simulink model "s20260910_config2torque_sim_pressure_torque"  (R2025a)
settings: Solver=VariableStepAuto  StartTime=0.0  StopTime=20  FixedStep=0.01  RelTol=1e-3  AbsTol=1e-3  EnableMultiTasking=on
undefined symbols (not defined in the file or in its folder): X, Y, Z
libraries: sm_lib x9, nesl_utility x4, cstblocks x2, snake_single_module_library_torque x1, slpidlib x1, simulink x1, snake_single_module_library_torque_multi x1
settings Model: Creator=dperera  LastModifiedBy=dperera
settings SolverCC: AutoScaleAbsTol=off  AlgebraicLoopSolver=TrustRegion  MaxZcPerStep=1.0
settings DataIOCC: LimitDataPoints=on  MaxDataPoints=10000
settings OptimizationCC: ReuseModelBlockBuffer=off  LifeSpan=inf
settings DebuggingCC: UnconnectedInputMsg=warning  UnconnectedOutputMsg=warning  UnconnectedLineMsg=warning  AllowSymbolicDim=off  SubsystemReferenceDiagnosticForUnitTest=warning  SFUnexpectedBacktrackingDiag=warning  SFNoUnconditionalDefaultTransitionDiag=warning  SFExecutionAtInitializationDiag=none  ArithmeticOperatorsInVariantConditions=warning
settings ModelReferenceCC: EnableRefExpFcnMdlSchedulingChecks=on
settings SFSimCC: SimUseLocalCustomCode=off  CustomCodeUndefinedFunction=UseInterfaceOnly
settings RTWCC: RTWUseLocalCustomCode=off  GPUComputeCapability=3.5  DLArmComputeVersion=19.05
settings CodeAppCC: StateflowObjectComments=on
settings GRTTargetCC: TargetLangStandard=C89/C90 (ANSI)
settings ConfigComp: CovMetricSettings=dw  CovSaveCumulativeToWorkspaceVar=on  CovSaveSingleToWorkspaceVar=on  CovExternalEMLEnable=off  CovSFcnEnable=off
settings SimscapeCC: SimscapeLogType=all  SimscapeLogSimulationStatistics=on  SimscapeLogDataHistory=10000.0

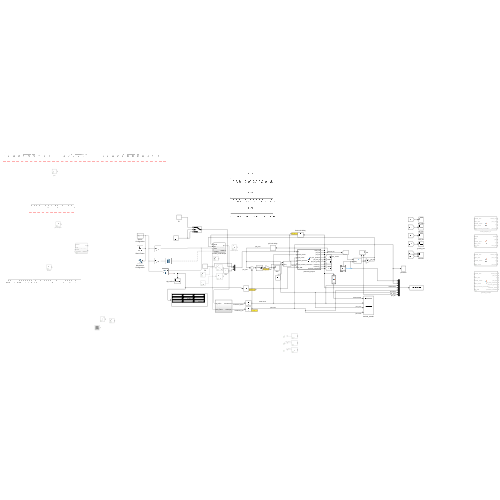
[thumbnail: Simulink's stored preview of the top-level diagram]
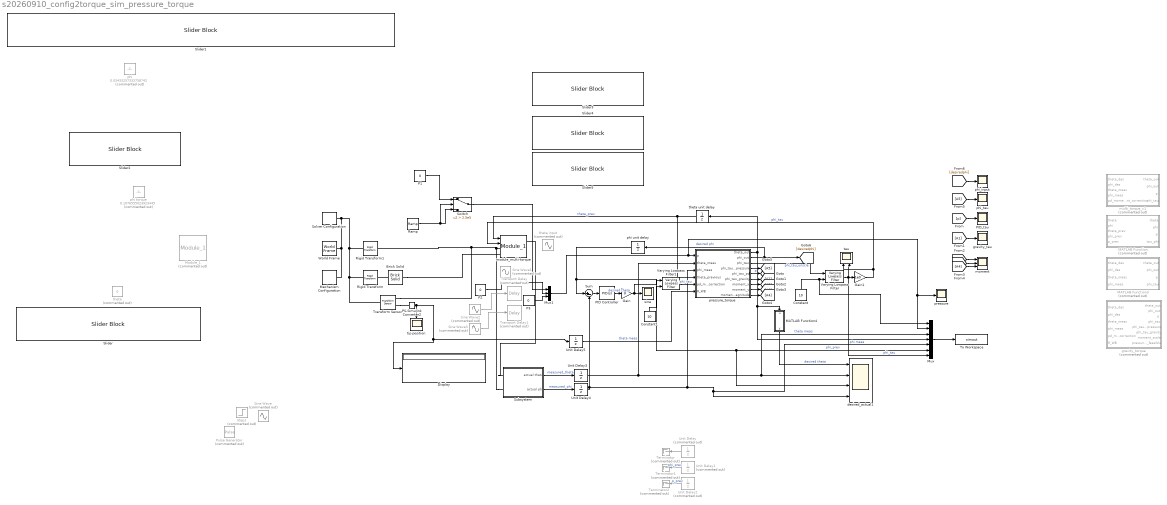
== system s20260910_config2torque_sim_pressure_torque ==
  Brick Solid : sm_lib/Body Elements/Brick Solid  BrickDimensions=[0.5 0.5 0.01]  BrickDimensionsUnits=m  ExportEntireGeometry=on  InertiaType=CalculateFromGeometry  BasedOnType=Density  Density=1000  DensityUnits=kg/m^3  Mass=1  MassUnits=kg  CenterOfMass=[0 0 0]  CenterOfMassUnits=m  MomentsOfInertia=[1 1 1]  MomentsOfInertiaUnits=kg*m^2  ProductsOfInertia=[0 0 0]  ProductsOfInertiaUnits=kg*m^2  GraphicType=FromGeometry  MarkerShape=Sphere  MarkerSize=10  GraphicVisPropType=SimpleVisualProperties  GraphicDiffuseColor=[0.5 0.5 0.5]  GraphicOpacity=1  GraphicSpecularColor=[0.5 0.5 0.5 1.0]  GraphicAmbientColor=[0.15 0.15 0.15 1.0]  GraphicEmissiveColor=[0.0 0.0 0.0 1.0]  GraphicShininess=75  DoExposeReferenceFrame=on  SerializedFrames=<Frames/>
  Constant : Constant  Value=10
  Constant1 : Constant  Value=10
  Display : Display
  Gain : Gain  Gain=0
  Gain1 : Gain  Gain=1e0
  MATLAB Function : MATLAB Function  Commented=on  TreatAsAtomicUnit=on
  MATLAB Function3 : MATLAB Function  Commented=on  TreatAsAtomicUnit=on
  MATLAB Function4 : MATLAB Function  TreatAsAtomicUnit=on
  Mechanism Configuration : sm_lib/Utilities/Mechanism Configuration  UniformGravity=Constant  GravityVector=[0 0 -9.80665]  GravityVectorUnits=m/s^2  LinearizationDelta=0.001  JointModeTransitionNonlinearIterations=2
  Module_1 : snake_single_module_library_torque/Module_1  Commented=on  SystemSampleTime=-1  VariantActivationTime=update diagram  EmptyChoice=off  PassThrough=off  PassThroughVariantControl=(default)  EmptyChoiceVariantControl=(default)  AllowFlexibleInterface=on  Latency=0  AutoFrameSizeCalculation=off
  Mux : Mux  Inputs=7
  Mux1 : Mux  Inputs=3
  P1 : Constant  Value=0
  P2 : Constant  Value=0
  P3 : Constant  Value=0
  PID Controller : slpidlib/PID Controller  Controller=PID  Form=Parallel  TimeDomain=Continuous-time  UseExternalTs=off  SampleTime=-1  IntegratorMethod=Forward Euler  FilterMethod=Forward Euler  ControllerParametersSource=internal  P=0.1  I=0.1  UseKiTs=off  D=0.0005  UseExternalDerivativeSource=off  N=100  UseFilter=on  TunerSelectOption=Frequency Response Based  InitialConditionSource=internal  InitialConditionForIntegrator=0  InitialConditionForFilter=0  DifferentiatorICPrevScaledInput=0  ExternalReset=none  TrackingMode=off  Kt=1  LimitOutput=on  SatLimitsSource=internal  UpperSaturationLimit=inf  LowerSaturationLimit=-inf  LinearizeAsGain=on  AntiWindupMode=back-calculation  Kb=1  LimitIntegrator=off  UpperIntegratorSaturationLimit=inf  LowerIntegratorSaturationLimit=-inf  POutMin=[]  POutMax=[]  IOutMin=[]  IOutMax=[]  DOutMin=[]  DOutMax=[]  NOutMin=[]  NOutMax=[]  SumOutMin=[]  SumOutMax=[]  SaturationOutMin=[]  SaturationOutMax=[]  PParamMin=[]  PParamMax=[]  IParamMin=[]  IParamMax=[]  DParamMin=[]  DParamMax=[]  NParamMin=[]  NParamMax=[]  KbParamMin=[]  KbParamMax=[]  KtParamMin=[]  KtParamMax=[]  KbOutMin=[]  KbOutMax=[]  KtOutMin=[]  KtOutMax=[]  IntegratorOutMin=[]  IntegratorOutMax=[]  FilterOutMin=[]  FilterOutMax=[]  SumI1OutMin=[]  SumI1OutMax=[]  SumI2OutMin=[]  SumI2OutMax=[]  SumI3OutMin=[]  SumI3OutMax=[]  SumI4OutMin=[]  SumI4OutMax=[]  SumDOutMin=[]  SumDOutMax=[]  DifferentiatorOutMin=[]  DifferentiatorOutMax=[]  FilterDiffOutCoefMin=[]  FilterDiffOutCoefMax=[]  ReciprocalOutMin=[]  ReciprocalOutMax=[]  SumDenOutMin=[]  SumDenOutMax=[]  SumNumOutMin=[]  SumNumOutMax=[]  DivideOutMin=[]  DivideOutMax=[]  UdiffTsProdOutMin=[]  UdiffTsProdOutMax=[]  NTsProdOutMin=[]  NTsProdOutMax=[]  UintegralTsProdOutMin=[]  UintegralTsProdOutMax=[]  UngainTsProdOutMin=[]  UngainTsProdOutMax=[]  ClampingZeroOutDataTypeStr=Inherit: Inherit via back propagation  ClampingZeroOutMin=[]  ClampingZeroOutMax=[]  FilterDenConstantOutDataTypeStr=Inherit: Inherit via back propagation  FilterDenConstantOutMin=[]  FilterDenConstantOutMax=[]  PCopyOutDataTypeStr=Inherit: Inherit via back propagation  PCopyOutMin=[]  PCopyOutMax=[]  NCopyOutDataTypeStr=Inherit: Inherit via back propagation  NCopyOutMin=[]  NCopyOutMax=[]  IntegratorContinuousStateAttributes=''  IntegratorStateMustResolveToSignalObject=off  IntegratorRTWStateStorageClass=Auto  FilterContinuousStateAttributes=''  FilterStateMustResolveToSignalObject=off  FilterRTWStateStorageClass=Auto  ParallelPVariant=InternalParameters  IdealPVariant=Disabled  IVariant=InternalParameters  DVariant=InternalParameters  IntegratorVariant=Continuous  SatVariant=Enabled  AWVariant=BackCalculation  PCopyVariant=Disabled  TRVariant=Disabled  FdbkBlocksVariant=Forward  IdealPFdbkVariant=Disabled  SatFdbkVariant=Disabled  DerivativeFilterVariant=ContFilter  NVariant=InternalParameters  NCopyVariant=Disabled  FilterICVariant=InternalICsFilter  IntegratorICVariant=InternalICs  ExternalResetVariant=Disabled  TRSumVariant=Passthrough  SumFdbkVariant=Disabled  SumVariant=Sum_PID  TsampFilterVariant=InternalTs  TsampNgainVariant=Passthrough  TsampIntegralVariant=Disabled_SignalSpec  ExternalSaturationOutDataTypeStr=Inherit: Same as second input  DerivativeSourceVariant=ErrorSignal  PreIntVariant=InternalPreInt
  PID_tau : Scope
      settings: ActiveDisplayYMinimum=-1  ActiveDisplayYMaximum=1  DataLoggingVariableName=ScopeData8
  PS-Simulink Converter2 : nesl_utility/PS-Simulink Converter  PhysicalDomain=network_engine_domain  SubClassName=ps_output  LeftPortType=input  RightPortType=output  PseudoPeriodic=off  Frequencies=[]  VectorFormat=inherit  Unit=inherit  AffineConversion=off
  Pulse Generator : DiscretePulseGenerator  Commented=on  PulseType=Time based  Amplitude=pi/3  Period=4  PulseWidth=50  PhaseDelay=1
  Ramp : simulink/Sources/Ramp  slope=50000  start=1  InitialOutput=10000
  Rigid Transform : sm_lib/Frames and Transforms/Rigid Transform  RotationMethod=None  FollAlignAxisA=+X  BaseAlignAxisA=+Y  FollAlignAxisB=+Y  BaseAlignAxisB=+Z  RotationStandardAxis=+Z  RotationAngle=0  RotationAngleUnits=deg  RotationArbitraryAxis=[0 0 1]  RotationSequenceAxes=FollowerAxes  RotationSequence=XYX  RotationSequenceAngles=[0 0 0]  RotationSequenceAnglesUnits=deg  RotationMatrix=[1 0 0;0 1 0;0 0 1]  Quaternion=[1 0 0 0]  TranslationMethod=StandardAxis  TranslationCartesianOffset=[0 0 0]  TranslationCartesianOffsetUnits=m  TranslationStandardAxis=+Z  TranslationStandardOffset=-0.03  TranslationStandardOffsetUnits=m  TranslationROffset=0  TranslationROffsetUnits=m  TranslationThetaOffset=0  TranslationThetaOffsetUnits=deg  TranslationZOffset=0  TranslationZOffsetUnits=m
  Rigid Transform1 : sm_lib/Frames and Transforms/Rigid Transform  RotationMethod=StandardAxis  FollAlignAxisA=+X  BaseAlignAxisA=+Y  FollAlignAxisB=+Y  BaseAlignAxisB=+Z  RotationStandardAxis=+X  RotationAngle=-pi/2  RotationAngleUnits=rad  RotationArbitraryAxis=[0 0 1]  RotationSequenceAxes=FollowerAxes  RotationSequence=XYX  RotationSequenceAngles=[0 0 0]  RotationSequenceAnglesUnits=deg  RotationMatrix=[1 0 0;0 1 0;0 0 1]  Quaternion=[1 0 0 0]  TranslationMethod=StandardAxis  TranslationCartesianOffset=[0 0 0]  TranslationCartesianOffsetUnits=m  TranslationStandardAxis=+Z  TranslationStandardOffset=0.3  TranslationStandardOffsetUnits=m  TranslationROffset=0  TranslationROffsetUnits=m  TranslationThetaOffset=0  TranslationThetaOffsetUnits=deg  TranslationZOffset=0  TranslationZOffsetUnits=m
  Sine Wave : Sin  Commented=on  Amplitude=pi/2-0.3  Bias=pi/2-0.3  Phase=3*pi/2  SampleTime=0
  Sine Wave1 : Sin  Commented=on  Amplitude=1.5e5  Bias=1.5e5  Phase=3*pi/2  SampleTime=0
  Sine Wave2 : Sin  Commented=on  Amplitude=1.5e5  Bias=1.5e5  Frequency=1.5  Phase=3*pi/2  SampleTime=0
  Sine Wave3 : Sin  Commented=on  Amplitude=1.5e5  Bias=1.5e5  Frequency=0.5  Phase=3*pi/2  SampleTime=0
  Slider : SliderBlock  ScaleMin=-3.14  ScaleMax=6
  Slider1 : SliderBlock  ScaleMax=3.14
  Slider2 : SliderBlock  ScaleMax=0.5
  Slider3 : SliderBlock  ScaleMax=350000
  Slider4 : SliderBlock  ScaleMax=350000
  Slider5 : SliderBlock  ScaleMax=350000
  Solver Configuration : nesl_utility/Solver Configuration  PhysicalDomain=network_engine_domain  SubClassName=solver  LeftPortType=input  RightPortType=generic  Tones=[]  Harmonics=[]  SimulateNoise=off  Profile=off  UseLocalSampling=off  EnableSwitchedLinearOptims=on  FrequencyDomain=off  UseCCode=off  RelTol=0.001  AbsTol=1e-06  MinStep=1e-09  ToWorkspace=off  RevertToSquareIcSolve=off  NumHomotopyIterations=100  PhasorMode=off  PhasorModeNumHarmonics=1  ConsistencySolver=NEWTON_XTOL_AFTER_FTOL  IndexReductionMethod=DerivativeReplacement  DoDC=off  ResidualTolerance=1e-09  ConsistencyTolSource=GLOBAL  ConsistencyAbsTol=0.001  ConsistencyRelTol=0.001  ConsistencyTolFactor=0.001  UseLocalSolver=off  LocalSolverChoice=NE_BACKWARD_EULER_ADVANCER  ResolveIndetEquations=on  FunctionEvalNumThread=1  LocalSolverSampleTime=0.001  DoFixedCost=off  MaxNonlinIter=3  MaxModeIter=2  ComputeImpulses=off  ImpulseIterations=2  LinearAlgebra=Sparse  LinearAlgebraNumThread=0  EquationFormulation=NE_TIME_EF  DelaysMemoryBudget=1024  AutomaticFiltering=on  FilteringTimeConstant=0.001  PartitionStorageMethod=AS_NEEDED  PartitionMemoryBudget=1024  PartitionMethod=FAST  MultibodyUseLocalSolver=off  MultibodyLocalSolverChoice=ODE1  MultibodyLocalSolverSampleTime=0.001
  Step1 : Step  Commented=on  After=pi/3  SampleTime=0
  Subsystem : Subsystem
  Sum : Sum  Inputs=|+-
  Switch : Switch  Criteria=u2 > Threshold  Threshold=2.5e5  SaturateOnIntegerOverflow=off  InputSameDT=off
  Terminator : Terminator  Commented=on
  Terminator1 : Terminator  Commented=on
  Terminator2 : Terminator  Commented=on
  To Workspace : ToWorkspace  VariableName=simout  SaveFormat=Timeseries  SampleTime=-1
      settings: Save2DSignal=2-D array (concatenate along first dimension)
  Transform Sensor : sm_lib/Frames and Transforms/Transform Sensor  MeasurementFrame=World  RotationSequence=XYX  SenseAngle=off  SenseAxis=off  SenseQ=off  SenseR=on  SenseRotationSequence=off  SenseOmegaX=off  SenseOmegaY=off  SenseOmegaZ=off  SenseOmega=off  SenseQDot=off  SenseRDot=off  SenseRotationSequenceDot=off  SenseAlphaX=off  SenseAlphaY=off  SenseAlphaZ=off  SenseAlpha=off  SenseQDDot=off  SenseRDDot=off  SenseX=off  SenseY=off  SenseZ=off  SenseXYZ=off  SenseRad=off  SenseAzim=off  SenseDist=off  SenseInc=off  SenseXDot=off  SenseYDot=off  SenseZDot=off  SenseXYZDot=off  SenseRadDot=off  SenseAzimDot=off  SenseDistDot=off  SenseIncDot=off  SenseXDDot=off  SenseYDDot=off  SenseZDDot=off  SenseXYZDDot=off  SenseRadDDot=off  SenseAzimDDot=off  SenseDistDDot=off  SenseIncDDot=off
  Transport Delay : TransportDelay  Commented=on  BufferSize=1024*3
  Transport Delay1 : TransportDelay  Commented=on  DelayTime=2  BufferSize=1024*3
  Unit Delay : UnitDelay  Commented=on  InitialCondition=[0]  SampleTime=-1  HasFrameUpgradeWarning=on
  Unit Delay1 : UnitDelay  Commented=on  InitialCondition=0.0001  SampleTime=-1  HasFrameUpgradeWarning=on
  Unit Delay2 : UnitDelay  Commented=on  InitialCondition=[0.0001;0.01;0.001]  SampleTime=-1  HasFrameUpgradeWarning=on
  Unit Delay3 : UnitDelay  InitialCondition=[0]  SampleTime=-1  HasFrameUpgradeWarning=on
  Unit Delay4 : UnitDelay  InitialCondition=0.0001  SampleTime=-1  HasFrameUpgradeWarning=on
  Unit Delay5 : UnitDelay  InitialCondition=[1 0 0;0 1 0;0 0 1]  SampleTime=-1  HasFrameUpgradeWarning=on
  Varying Lowpass Filter : cstblocks/Linear Parameter Varying/Varying Lowpass Filter  N=1
  Varying Lowpass Filter1 : cstblocks/Linear Parameter Varying/Varying Lowpass Filter  N=1
  World Frame : sm_lib/Frames and Transforms/World Frame
  desired_actual1 : Scope  NumInputPorts=4
      settings: ActiveDisplayYMinimum=-3.92699081698724  ActiveDisplayYMaximum=3.9269908169872312  DataLoggingVariableName=ScopeData7
  gravity_tau : Scope
      settings: ActiveDisplayYMinimum=-0.011322390478246933  ActiveDisplayYMaximum=0.10190151430422241  DataLoggingVariableName=ScopeData9
  gravity_torque : MATLAB Function  Commented=on  TreatAsAtomicUnit=on
  module_multi-torque : snake_single_module_library_torque_multi/Module_1  SystemSampleTime=-1  VariantActivationTime=update diagram  EmptyChoice=off  PassThrough=off  PassThroughVariantControl=(default)  EmptyChoiceVariantControl=(default)  AllowFlexibleInterface=on  Latency=0  AutoFrameSizeCalculation=off
  "moment " : Scope  NumInputPorts=3
      settings: ActiveDisplayYMinimum=-0.80428663695757552  ActiveDisplayYMaximum=1.2004762929952861  DataLoggingVariableName=ScopeData10
  multi_torque_v1 : MATLAB Function  Commented=on  TreatAsAtomicUnit=on
  phi : Constant  Commented=on  Value=0.03433257333758742
  phi torque : Constant  Commented=on  Value=0.1076555023923445
  phi unit delay : UnitDelay  InitialCondition=[0]  SampleTime=-1  HasFrameUpgradeWarning=on
  phi_input : Scope
      settings: ActiveDisplayYMinimum=-0.36834079509334744  ActiveDisplayYMaximum=3.3160671558401278  DataLoggingVariableName=ScopeData3
  phi_tau : Scope
      settings: ActiveDisplayYMinimum=-0.0992891016231981  ActiveDisplayYMaximum=0.63745599903013284  DataLoggingVariableName=ScopeData11
  pressure : Scope
      settings: ActiveDisplayYMinimum=-31249.999999999643  ActiveDisplayYMaximum=281249.99999999686  DataLoggingVariableName=ScopeData4
  pressure_torque : MATLAB Function  TreatAsAtomicUnit=on
  sine : Scope
      settings: ActiveDisplayYMinimum=-0.21170008314097447  ActiveDisplayYMaximum=0.0761701023793398  DataLoggingVariableName=ScopeData2
  tau : Scope  NumInputPorts=2
      settings: ActiveDisplayYMinimum=-0.18342543363642283  ActiveDisplayYMaximum=0.62410632446902137
  theta : Constant  Commented=on  Value=0
  theta input : Sin  Commented=on  Amplitude=pi-0.1  Frequency=0.1  SampleTime=0
  theta unit delay : UnitDelay  InitialCondition=[0]  SampleTime=-1  HasFrameUpgradeWarning=on
  tip position : Scope
      settings: ActiveDisplayYMinimum=-1.2500000000000002  ActiveDisplayYMaximum=1.2500000000000004  DataLoggingVariableName=ScopeData5
  wires:
  MATLAB Function4/1(y) -> desired_actual1/1  "desired theta"
  Gain1/1 -> tau/1, module_multi-torque/2  "phi_tau"
  pressure_torque/2(phi_out) -> phi unit delay/1, [desiredphi]  "desired phi"
  Subsystem/1(actual theta) -> Unit Delay3/1  "measured_theta"
  Subsystem/2(actual phi) -> Unit Delay4/1  "measured_phi"
  Mux/1 -> To Workspace/1
  PID Controller/1 -> Gain/1  "desired theta"
  Unit Delay/1 -> Terminator/1
  Unit Delay1/1 -> Terminator1/1  "phi_prev"
  Unit Delay2/1 -> Terminator2/1  "p_prev"
  Unit Delay3/1 -> desired_actual1/2, Mux/3, pressure_torque/2(theta_meas)  "theta meas"
  Unit Delay4/1 -> desired_actual1/4, Mux/5, pressure_torque/3(phi_meas), Sum/2  "phi meas"
  Sum/1 -> PID Controller/1
  pressure_torque/3(phi_tau) -> Varying Lowpass Filter/1  "phi_tau_unscle"
  Varying Lowpass Filter/1 -> Mux/7, Gain1/1, tau/2  "phi_tau"
  Constant/1 -> Varying Lowpass Filter/2, Mux/1
  PS-Simulink Converter2/1 -> Display/1, Unit Delay5/1, tip position/1
  pressure_torque/1(theta_out) -> theta unit delay/1, MATLAB Function4/1(u), Mux/4
  Unit Delay5/1 -> pressure_torque/6(R_WB)  "theta meas"
  theta unit delay/1 -> pressure_torque/4(theta_previous), module_multi-torque/1  "theta_prev"
  pressure_torque/5(phi_tau_pd) -> [p]  "p"
  [p] -> PID_tau/1
  pressure_torque/6(phi_tau_gravity) -> [A1]
  [A1] -> gravity_tau/1
  pressure_torque/7(moment_x) -> [A2]
  [A2] -> "moment "/1
  pressure_torque/8(moment_y) -> [A3]
  [A3] -> "moment "/2
  pressure_torque/9(moment_magnitude) -> [A4]
  [A4] -> "moment "/3
  pressure_torque/4(phi_tau_pressure) -> [A5]
  [A5] -> phi_tau/1
  [desiredphi] -> phi_input/1
  Sine Wave2/1 -> Transport Delay/1
  Mux1/1 -> Mux/2, pressure/1, pressure_torque/1(p)
  phi unit delay/1 -> Sum/1, Mux/6, desired_actual1/3  "phi_prev"
  Sine Wave3/1 -> Transport Delay1/1
  Varying Lowpass Filter1/1 -> pressure_torque/5(pd_moment_correction)  "phi_tau"
  Constant1/1 -> Varying Lowpass Filter1/2
  P3/1 -> Mux1/3
  P2/1 -> Mux1/2
  Ramp/1 -> Switch/2, Switch/3
  P1/1 -> Switch/1
  Switch/1 -> Mux1/1
  Gain/1 -> Varying Lowpass Filter1/1, sine/1
  connections:
  World Frame/RConn1 -- Transform Sensor/LConn1 -- Rigid Transform/LConn1 -- Rigid Transform1/LConn1 -- Solver Configuration/RConn1 -- Mechanism Configuration/RConn1
  Brick Solid/RConn1 -- Rigid Transform/RConn1
  Subsystem/LConn2 -- Transform Sensor/RConn1 -- Rigid Transform1/RConn1 -- module_multi-torque/LConn1
  Brick Solid/LConn1 -- module_multi-torque/LConn2
  Subsystem/LConn1 -- module_multi-torque/RConn1
  Transform Sensor/RConn2 -- PS-Simulink Converter2/LConn1

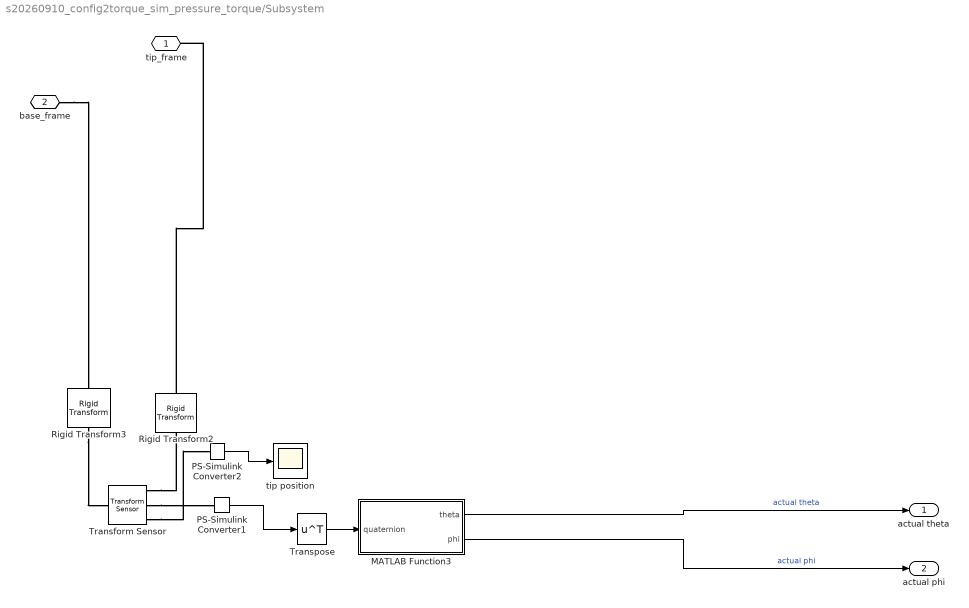
== system s20260910_config2torque_sim_pressure_torque/Subsystem ==
  MATLAB Function3 : MATLAB Function  TreatAsAtomicUnit=on
  PS-Simulink Converter1 : nesl_utility/PS-Simulink Converter  PhysicalDomain=network_engine_domain  SubClassName=ps_output  LeftPortType=input  RightPortType=output  PseudoPeriodic=off  Frequencies=[]  VectorFormat=inherit  Unit=inherit  AffineConversion=off
  PS-Simulink Converter2 : nesl_utility/PS-Simulink Converter  PhysicalDomain=network_engine_domain  SubClassName=ps_output  LeftPortType=input  RightPortType=output  PseudoPeriodic=off  Frequencies=[]  VectorFormat=inherit  Unit=inherit  AffineConversion=off
  Rigid Transform2 : sm_lib/Frames and Transforms/Rigid Transform  RotationMethod=RotationSequence  FollAlignAxisA=+X  BaseAlignAxisA=+Y  FollAlignAxisB=+Y  BaseAlignAxisB=+Z  RotationStandardAxis=+Z  RotationAngle=pi  RotationAngleUnits=rad  RotationArbitraryAxis=[0 0 1]  RotationSequenceAxes=FollowerAxes  RotationSequence=XZY  RotationSequenceAngles=[-pi/2 pi 0]  RotationSequenceAnglesUnits=rad  RotationMatrix=[1 0 0;0 1 0;0 0 1]  Quaternion=[1 0 0 0]  TranslationMethod=None  TranslationCartesianOffset=[0 0 0]  TranslationCartesianOffsetUnits=m  TranslationStandardAxis=+Z  TranslationStandardOffset=-0.5  TranslationStandardOffsetUnits=m  TranslationROffset=0  TranslationROffsetUnits=m  TranslationThetaOffset=0  TranslationThetaOffsetUnits=deg  TranslationZOffset=0  TranslationZOffsetUnits=m
  Rigid Transform3 : sm_lib/Frames and Transforms/Rigid Transform  RotationMethod=RotationSequence  FollAlignAxisA=+X  BaseAlignAxisA=+Y  FollAlignAxisB=+Y  BaseAlignAxisB=+Z  RotationStandardAxis=+Z  RotationAngle=pi  RotationAngleUnits=rad  RotationArbitraryAxis=[0 0 1]  RotationSequenceAxes=FollowerAxes  RotationSequence=YXZ  RotationSequenceAngles=[pi -pi/2 0]  RotationSequenceAnglesUnits=rad  RotationMatrix=[1 0 0;0 1 0;0 0 1]  Quaternion=[1 0 0 0]  TranslationMethod=None  TranslationCartesianOffset=[0 0 0]  TranslationCartesianOffsetUnits=m  TranslationStandardAxis=+Z  TranslationStandardOffset=-0.5  TranslationStandardOffsetUnits=m  TranslationROffset=0  TranslationROffsetUnits=m  TranslationThetaOffset=0  TranslationThetaOffsetUnits=deg  TranslationZOffset=0  TranslationZOffsetUnits=m
  Transform Sensor : sm_lib/Frames and Transforms/Transform Sensor  MeasurementFrame=Follower  RotationSequence=XYZ  SenseAngle=off  SenseAxis=off  SenseQ=on  SenseR=off  SenseRotationSequence=off  SenseOmegaX=off  SenseOmegaY=off  SenseOmegaZ=off  SenseOmega=off  SenseQDot=off  SenseRDot=off  SenseRotationSequenceDot=off  SenseAlphaX=off  SenseAlphaY=off  SenseAlphaZ=off  SenseAlpha=off  SenseQDDot=off  SenseRDDot=off  SenseX=off  SenseY=off  SenseZ=off  SenseXYZ=on  SenseRad=off  SenseAzim=off  SenseDist=off  SenseInc=off  SenseXDot=off  SenseYDot=off  SenseZDot=off  SenseXYZDot=off  SenseRadDot=off  SenseAzimDot=off  SenseDistDot=off  SenseIncDot=off  SenseXDDot=off  SenseYDDot=off  SenseZDDot=off  SenseXYZDDot=off  SenseRadDDot=off  SenseAzimDDot=off  SenseDistDDot=off  SenseIncDDot=off
  Transpose : Math  Operator=transpose
  tip position : Scope
      settings: ActiveDisplayYMinimum=-0.036250000065594909  ActiveDisplayYMaximum=0.32625000000729432  DataLoggingVariableName=ScopeData6
  tip_frame : PMIOPort  Side=Left
  base_frame : PMIOPort  Port=2  Side=Left
  actual theta : Outport
  actual phi : Outport  Port=2
  wires:
  PS-Simulink Converter1/1 -> Transpose/1
  Transpose/1 -> MATLAB Function3/1(quaternion)
  MATLAB Function3/2(phi) -> actual phi/1  "actual phi"
  PS-Simulink Converter2/1 -> tip position/1
  MATLAB Function3/1(theta) -> actual theta/1  "actual theta"
  connections:
  Transform Sensor/RConn1 -- Rigid Transform2/RConn1
  Transform Sensor/RConn2 -- PS-Simulink Converter1/LConn1
  Rigid Transform3/RConn1 -- Transform Sensor/LConn1
  Transform Sensor/RConn3 -- PS-Simulink Converter2/LConn1
  base_frame/RConn1 -- Rigid Transform3/LConn1
  Rigid Transform2/LConn1 -- tip_frame/RConn1

== matlab function s20260910_config2torque_sim_pressure_torque/MATLAB Function ==
  data: theta input; theta output; phi input; theta_prev input; phi_prev input; p_prev input; phi output; p output; tau_phi output
function [theta, phi, p, tau_phi] = fcn(theta, phi, theta_prev, phi_prev, p_prev)
%#codegen 
% 
% This function computes torque required for the
% 
A = pi * (0.013/2)^2;
r = 0.013;
K = 0.00001;
N = 30;
L = 0.29;
l = L/N;

J_angle = f20260427_3_pressure2config_Jacobian(p_prev, A, K, r);
J_inv = pinv(J_angle);
% p = p_mat(:, i) + J_inv*([theta(i+1); phi(i+1)]-[frw(1,i); frw(2,i)]);
p = p_prev + J_inv*([theta; phi]-[theta_prev; phi_prev]);
% p = m20260427_5_PositivePressures(p);


[f, my, mx, ~, ~] = pressure2force_moment_config(p, A, r, K);
W = [mx; my; 0.0; 0.0; 0.0; f];
J = completeArm_Jacobian(theta_prev, phi_prev, l, N);

tau = J' * W;
tau_phi = tau(2);

== matlab function s20260910_config2torque_sim_pressure_torque/pressure_torque ==
  data: p input; theta_meas input; phi_meas input; theta_out output; theta_previous input; phi_out output; phi_tau output; phi_tau_pressure output; phi_tau_pd output; pd_moment_correction input; R_WB input; phi_tau_gravity output; moment_x output; moment_y output; moment_magnitude output
function [theta_out, phi_out, phi_tau, ...
          phi_tau_pressure, phi_tau_pd, phi_tau_gravity, ...
          moment_x, moment_y, moment_magnitude] = ...
    fcn(p, theta_meas, phi_meas, theta_previous, ...
        pd_moment_correction, R_WB)

%#codegen
%
% Pressure-to-torque calculation for the rigid-link approximation.
%
% Inputs:
%   p                    : muscle pressures [3x1] [Pa]
%   theta_meas           : measured bending direction [rad]
%   phi_meas             : measured total bending angle [rad]
%   theta_previous       : previous theta_out from a Unit Delay [rad]
%   pd_moment_correction : PD/PID bending-moment correction [N*m]
%   R_WB                 : rotation supplied by Simscape [3x3]
%
% Outputs:
%   theta_out            : pressure-derived bending direction [rad]
%   phi_out              : pressure-derived static phi reference [rad]
%   phi_tau              : final first-phi torque for each interval [29x1]
%   phi_tau_pressure     : pressure contribution [29x1]
%   phi_tau_pd           : PD/PID contribution [29x1]
%   phi_tau_gravity      : gravity compensation contribution [29x1]
%   moment_x             : pressure-generated x moment [N*m]
%   moment_y             : pressure-generated y moment [N*m]
%   moment_magnitude     : resultant pressure moment [N*m]

%% Model parameters

A = pi*(0.013/2)^2;     % Effective muscle area [m^2]
r = 0.013;              % Muscle radial offset [m]
K = 0.19223750;         % Continuum bending stiffness [N*m/rad]

N = 29;                 % Number of rigid-link intervals
L = 0.29;               % Arm length [m]
l = L/N;                % Length of one interval [m]

% Update this value to match the mass assigned to one moving disk
% in the Simscape model.
module_mass = 0.100;              % Total module mass [kg]
number_disks = N + 1;             % 30 physical disks
disk_mass = module_mass/number_disks;

%% Pressure-generated bending moments

Ar = A*r;

p1 = p(1);
p2 = p(2);
p3 = p(3);

moment_x = Ar*sqrt(3)*(p2 - p3)/2;
moment_y = Ar*(p2 + p3 - 2*p1)/2;

moment_magnitude = sqrt(moment_x^2 + moment_y^2);

%% Calculate the pressure-derived theta

moment_threshold = 1e-8;

if moment_magnitude > moment_threshold

    % The moment convention is:
    %
    % Mx = -M*sin(theta)
    % My =  M*cos(theta)

    theta_raw = atan2(-moment_x, moment_y);

    % Select the equivalent theta nearest to the previous command.
    % This prevents unnecessary jumps between -pi and +pi.
    theta_difference = atan2( ...
        sin(theta_raw - theta_previous), ...
        cos(theta_raw - theta_previous));

    theta_out = theta_previous + theta_difference;

else

    % The bending direction is undefined when the resultant moment is zero.
    theta_out = theta_previous;

end

%% Static phi reference generated by pressure

% This is the nominal static relation M = K*phi.
phi_out = moment_magnitude/K;

%% Configuration used for the Jacobian and gravity calculations

% Theta estimated from the tip pose is unreliable near phi = 0.
phi_threshold = 1e-6;

if abs(phi_meas) < phi_threshold
    theta_for_model = theta_out;
else
    theta_for_model = theta_meas;
end

phi_for_model = phi_meas;

%% Pressure-generated wrench

% Moment-only wrench.
%
% The axial pressure force is intentionally excluded because the
% backbone supports the axial load in the present approximation.
W_pressure = [moment_x;
              moment_y;
              0;
              0;
              0;
              0];

%% PD/PID moment correction

% Apply the controller correction along the current bending direction.
%
% Positive correction increases bending.
% Negative correction produces a restoring moment.

moment_x_pd = -pd_moment_correction*sin(theta_out);
moment_y_pd =  pd_moment_correction*cos(theta_out);

W_pd = [moment_x_pd;
        moment_y_pd;
        0;
        0;
        0;
        0];

%% Pressure and PD/PID joint torques

J = completeArm_Jacobian( ...
    theta_for_model, phi_for_model, l, N);

tau_pressure_all = J.'*W_pressure;
tau_pd_all       = J.'*W_pd;

% Select the first phi joint from each rigid-link interval.
%
% Complete joint order:
%   theta, phi_1, phi_2, -theta
%
% MATLAB indices of the first phi joints:
%   2, 6, 10, ..., 114

phi_tau_pressure = zeros(N,1);
phi_tau_pd       = zeros(N,1);

for i = 1:N

    complete_joint_index = 2 + 4*(i - 1);

    phi_tau_pressure(i) = ...
        tau_pressure_all(complete_joint_index);

    phi_tau_pd(i) = ...
        tau_pd_all(complete_joint_index);

end

%% Convert world gravity into the kinematic arm frame

% Simscape gravity vector
gravity_world = [0;
                 0;
                -9.80665];

% Fixed alignment between:
%   K: the kinematic frame, where the undeformed arm extends along +z
%   M: the nominal Simscape frame, where the arm is horizontal along +y
R_MK = [1  0  0;
        0  0  1;
        0 -1  0];       % Rx(-pi/2)

% Complete transformation from the kinematic frame to the world frame
R_WK = R_WB*R_MK;

% Gravity expressed in the kinematic frame
gravity_kinematic = R_WK.'*gravity_world;

% Gravity force acting on one moving disk
gravity_force_disk = disk_mass*gravity_kinematic;

%% Construct the measured rigid-link geometry

% Each interval contains:
%
% Rz(theta) -> Ry(phi/(2N)) -> Tz(l)
% -> Ry(phi/(2N)) -> Rz(-theta)

alpha = phi_for_model/(2*N);

ct = cos(theta_for_model);
st = sin(theta_for_model);

ca = cos(alpha);
sa = sin(alpha);

Rz_theta = [ct -st  0;
            st  ct  0;
             0   0  1];

Rz_minus_theta = [ ct  st  0;
                  -st  ct  0;
                    0   0  1];

Ry_alpha = [ ca  0  sa;
              0  1   0;
            -sa  0  ca];

unit_y = [0; 1; 0];
translation_local = [0; 0; l];

% Two phi joints per interval are retained internally.
number_phi_joints = 2*N;

phi_joint_axis   = zeros(3,number_phi_joints);
phi_joint_origin = zeros(3,number_phi_joints);

% Position of each moving downstream disk
disk_position = zeros(3,N);

R_current = eye(3);
position_current = zeros(3,1);

for i = 1:N

    first_phi_index  = 2*i - 1;
    second_phi_index = 2*i;

    % First rotation: Rz(theta)
    R_after_theta = R_current*Rz_theta;

    % First phi joint
    phi_joint_axis(:,first_phi_index) = ...
        R_after_theta*unit_y;

    phi_joint_origin(:,first_phi_index) = ...
        position_current;

    % First half-phi rotation
    R_after_phi_1 = R_after_theta*Ry_alpha;

    % Translation to the next disk
    position_next = ...
        position_current + R_after_phi_1*translation_local;

    % Second phi joint is located at the next disk
    phi_joint_axis(:,second_phi_index) = ...
        R_after_phi_1*unit_y;

    phi_joint_origin(:,second_phi_index) = ...
        position_next;

    % Disk center is currently approximated by its frame origin.
    disk_position(:,i) = position_next;

    % Complete the second half-phi and -theta rotations
    R_after_phi_2 = R_after_phi_1*Ry_alpha;

    R_current = R_after_phi_2*Rz_minus_theta;
    position_current = position_next;

end

%% Calculate gravity torque at every phi joint

phi_gravity_load_all = zeros(number_phi_joints,1);

for j = 1:number_phi_joints

    % Identify the interval containing this phi joint
    interval_index = floor((j - 1)/2) + 1;

    gravity_load_j = 0;

    % Add gravity moments produced by all downstream moving disks
    for k = interval_index:N

        joint_to_disk = ...
            disk_position(:,k) - phi_joint_origin(:,j);

        gravity_moment_at_joint = ...
            cross(joint_to_disk, gravity_force_disk);

        gravity_load_j = gravity_load_j + ...
            phi_joint_axis(:,j).'*gravity_moment_at_joint;

    end

    phi_gravity_load_all(j) = gravity_load_j;

end

% Compensation torque must oppose the gravity load torque.
phi_gravity_compensation_all = -phi_gravity_load_all;

%% Select the first phi-joint gravity torque from each interval

phi_tau_gravity = zeros(N,1);

for i = 1:N

    first_phi_index = 2*i - 1;

    phi_tau_gravity(i) = ...
        phi_gravity_compensation_all(first_phi_index);

end

%% Final torque command

phi_tau = ...
    phi_tau_pressure + ...
    phi_tau_pd + ...
    phi_tau_gravity;

end

== matlab function s20260910_config2torque_sim_pressure_torque/Subsystem/MATLAB Function3 ==
  data: quaternion input; theta output; phi output
function [theta, phi] = IMU2Config(quaternion)
%#codegen
T = quat2rotm(quaternion);

theta= wrapToPi(atan2(T(2,3),T(1,3)));
phi= (acos(T(3,3)));

end

== matlab function s20260910_config2torque_sim_pressure_torque/MATLAB Function4 ==
  data: u input; y output
function y = fcn(u)
%$codegen
y = wrapToPi(u);

== matlab function s20260910_config2torque_sim_pressure_torque/MATLAB Function3 ==
  data: theta_des input; theta_out output; phi_des input; theta_meas input; phi_meas input; phi_out output; p output; phi_tau output
function [theta_out, phi_out, p, phi_tau] = ...
    fcn(theta_des, phi_des, theta_meas, phi_meas)

%#codegen
%
% Inputs:
%   theta_des  : desired bending direction [rad]
%   phi_des    : desired total bending angle [rad]
%   theta_meas : measured bending direction [rad]
%   phi_meas   : measured total bending angle [rad]
%
% Outputs:
%   theta_out  : desired theta passed to the theta position controller
%   phi_out    : desired phi for logging
%   p          : calculated muscle pressures [Pa]
%   tau_phi    : first phi-joint torque [N*m]

%% Model parameters

A = pi*(0.013/2)^2;     % Muscle area [m^2]
r = 0.013;              % Muscle radial offset [m]
K = 0.19223750;            % Continuum bending stiffness [N*m/rad]

N = 29;                 % Number of rigid-link intervals
L = 0.29;               % Arm length [m]
l = L/N;                % Link length [m]

theta_out = theta_des;
phi_out = phi_des;

%% Select the common pressure

% Maximum expected bending angle
phi_max = pi;

% Minimum common pressure required to prevent negative pressures.
% The factor 1.10 adds a 10% margin.
p_common = 1.10*(2*K*phi_max)/(3*A*r);

%% Direct configuration-to-pressure mapping

% Desired bending moments
my_des = K*phi_des*cos(theta_des);
mx_des = -K*phi_des*sin(theta_des);

Ar = A*r;

p1 = p_common - 2*my_des/(3*Ar);

p2 = p_common ...
   + my_des/(3*Ar) ...
   + mx_des/(sqrt(3)*Ar);

p3 = p_common ...
   + my_des/(3*Ar) ...
   - mx_des/(sqrt(3)*Ar);

p = [p1; p2; p3];

% Numerical protection. Adding the same pressure to all three muscles
% does not change the desired bending moments.
% minimum_pressure = min(p);
% 
% if minimum_pressure < 0
%     p = p - minimum_pressure;
% end

%% Calculate the tip wrench

% Corrected axial force
force_z = A*sum(p);

% Recalculate moments from the resulting pressures
moment_y = -(A*r*(-p(2) - p(3) + 2*p(1)))/2;
moment_x = A*r*sqrt(3)*(p(2) - p(3))/2;

% Tip-frame wrench:
% [Mx; My; Mz; Fx; Fy; Fz]
W = [moment_x;
     moment_y;
     0;
     0;
     0;
     0];

%% Calculate joint torques at the measured configuration

% Theta from a tip-pose estimator may be undefined when phi is almost zero.
% In that small region, use the commanded theta.
if abs(phi_meas) < 1e-6
    theta_for_J = theta_des;
else
    theta_for_J = theta_meas;
end

J = completeArm_Jacobian( ...
    theta_for_J, phi_meas, l, N);

tau = J.'*W;

% First phi joint. This preserves your current common-torque experiment.
phi_tau = tau(2);

end

== matlab function s20260910_config2torque_sim_pressure_torque/multi_torque_v1 ==
  data: theta_des input; theta_out output; phi_des input; theta_meas input; phi_meas input; phi_out output; p output; phi_tau output; pd_moment_correction input
function [theta_out, phi_out, p, phi_tau] = ...
    fcn(theta_des, phi_des, theta_meas, phi_meas, pd_moment_correction)

%#codegen
%
% Inputs:
%   theta_des  : desired bending direction [rad]
%   phi_des    : desired total bending angle [rad]
%   theta_meas : measured bending direction [rad]
%   phi_meas   : measured total bending angle [rad]
%
% Outputs:
%   theta_out  : desired theta passed to the theta position controller
%   phi_out    : desired phi for logging
%   p          : calculated muscle pressures [Pa]
%   tau_phi    : first phi-joint torque [N*m]

%% Model parameters

A = pi*(0.013/2)^2;     % Muscle area [m^2]
r = 0.013;              % Muscle radial offset [m]
K = 0.19223750;            % Continuum bending stiffness [N*m/rad]

N = 29;                 % Number of rigid-link intervals
L = 0.29;               % Arm length [m]
l = L/N;                % Link length [m]

theta_out = theta_des;
phi_out = phi_des;


%% Desired bending moments

% my_des = K*phi_des*cos(theta_des);
% mx_des = -K*phi_des*sin(theta_des);

bending_moment_cmd = ...
    K*phi_des + pd_moment_correction;

my_des = bending_moment_cmd*cos(theta_des);
mx_des = -bending_moment_cmd*sin(theta_des);

%% Null-space pressure allocation

Ar = A*r;

% Differential pressures producing the desired moments.
% Their sum is zero.
p_delta = [ ...
    -2*my_des/(3*Ar);
     my_des/(3*Ar) + mx_des/(sqrt(3)*Ar);
     my_des/(3*Ar) - mx_des/(sqrt(3)*Ar)];

% Physical pressure limits
p_min = 0;          % [Pa]
p_max = 350000;     % 3.5 bar [Pa]

% Range of common pressure that satisfies all pressure limits
p_common_min = p_min - min(p_delta);
p_common_max = p_max - max(p_delta);

if p_common_min <= p_common_max

    % Desired bending moment is feasible.
    % Midpoint gives equal margin from the upper and lower limits.
    p_common = 0.5*(p_common_min + p_common_max);

    p = p_delta + p_common;

    moment_scale = 1.0;
    pressure_feasible = true;

else

    % Requested moment cannot be generated within the pressure limits.
    % Scale the differential pressures while preserving theta.
    pressure_span = max(p_delta) - min(p_delta);

    if pressure_span > 1e-12
        moment_scale = (p_max - p_min)/pressure_span;
    else
        moment_scale = 1.0;
    end

    p_delta = moment_scale*p_delta;

    % Recalculate the feasible common-pressure interval
    p_common_min = p_min - min(p_delta);
    p_common_max = p_max - max(p_delta);

    p_common = 0.5*(p_common_min + p_common_max);

    p = p_delta + p_common;

    pressure_feasible = false;

end

%% Recalculate achievable moments from allocated pressures

moment_y = -(A*r*(-p(2) - p(3) + 2*p(1)))/2;
moment_x = A*r*sqrt(3)*(p(2) - p(3))/2;

%% Moment-only tip wrench

W = [moment_x;
     moment_y;
     0;
     0;
     0;
     0];

%% Joint torque calculation

if abs(phi_meas) < 1e-6
    theta_for_J = theta_des;
else
    theta_for_J = theta_meas;
end

J = completeArm_Jacobian( ...
    theta_for_J, phi_meas, l, N);

tau = J.'*W;

ii = 1:1:N;
idx = 2+4*(ii-1);

phi_tau = tau(idx);

end

== matlab function s20260910_config2torque_sim_pressure_torque/gravity_torque ==
  data: theta_des input; theta_out output; phi_des input; theta_meas input; phi_meas input; phi_out output; p output; phi_tau output; pd_moment_correction input; R_WB input; phi_tau_pressure output; phi_tau_gravity output; moment_scale output; pressure_feasible output
function [theta_out, phi_out, p, phi_tau, ...
          phi_tau_pressure, phi_tau_gravity, ...
          moment_scale, pressure_feasible] = ...
    fcn(theta_des, phi_des, theta_meas, phi_meas, ...
        pd_moment_correction, R_WB)

%#codegen
%
% Inputs:
%   theta_des            : desired bending direction [rad]
%   phi_des              : desired total bending angle [rad]
%   theta_meas           : measured bending direction [rad]
%   phi_meas             : measured total bending angle [rad]
%   pd_moment_correction : PD correction added to bending moment [N*m]
%   R_WB                 : rotation matrix from arm base to world [3x3]
%
%                           v_world = R_WB*v_base
%
% Outputs:
%   theta_out       : desired theta for theta position controller [rad]
%   phi_out         : desired phi for logging [rad]
%   p               : allocated muscle pressures [3x1], Pa
%   phi_tau         : final torque for all 58 phi joints [58x1], N*m
%   phi_tau_pressure: pressure-generated phi-joint torque [58x1], N*m
%   phi_tau_gravity : gravity-compensation torque [58x1], N*m
%   moment_scale    : pressure-allocation moment scaling factor
%   pressure_feasible: true if the requested moment is feasible
%
% phi_tau ordering:
%   phi_tau(1)  = interval 1, Phi1
%   phi_tau(2)  = interval 1, Phi2
%   phi_tau(3)  = interval 2, Phi1
%   phi_tau(4)  = interval 2, Phi2
%   ...
%   phi_tau(57) = interval 29, Phi1
%   phi_tau(58) = interval 29, Phi2

%% Model parameters

A = pi*(0.013/2)^2;     % Effective muscle area [m^2]
r = 0.013;              % Muscle radial offset [m]
K = 0.19223750;         % Continuum bending stiffness [N*m/rad]

N = 29;                 % Number of rigid-link intervals
L = 0.29;               % Arm length [m]
l = L/N;                % Link length [m]

number_phi_joints = 2*N;

% Total module mass is assumed to be 0.100 kg over 30 disks.
% The base disk is fixed but each moving disk retains the same mass.
disk_mass = 0.100/30;   % [kg]

theta_out = theta_des;
phi_out = phi_des;

%% Desired bending moments

% The PD controller modifies the commanded bending moment.
bending_moment_cmd = K*phi_des + pd_moment_correction;

my_des =  bending_moment_cmd*cos(theta_des);
mx_des = -bending_moment_cmd*sin(theta_des);

%% Null-space pressure allocation

Ar = A*r;

% Differential-pressure component. Its sum is zero, so adding a common
% pressure does not change the bending moments.
p_delta = [ ...
    -2*my_des/(3*Ar);
     my_des/(3*Ar) + mx_des/(sqrt(3)*Ar);
     my_des/(3*Ar) - mx_des/(sqrt(3)*Ar)];

p_min = 0;              % Minimum pressure [Pa]
p_max = 350000;         % Maximum pressure: 3.5 bar [Pa]

p_common_min = p_min - min(p_delta);
p_common_max = p_max - max(p_delta);

if p_common_min <= p_common_max

    % Requested bending moment is feasible.
    p_common = 0.5*(p_common_min + p_common_max);

    p = p_delta + p_common;

    moment_scale = 1.0;
    pressure_feasible = true;

else

    % Scale the differential pressures while preserving theta.
    pressure_span = max(p_delta) - min(p_delta);

    if pressure_span > 1e-12
        moment_scale = (p_max - p_min)/pressure_span;
    else
        moment_scale = 1.0;
    end

    p_delta = moment_scale*p_delta;

    p_common_min = p_min - min(p_delta);
    p_common_max = p_max - max(p_delta);

    p_common = 0.5*(p_common_min + p_common_max);

    p = p_delta + p_common;

    pressure_feasible = false;

end

%% Recalculate the achievable moments

moment_y = -(A*r*(-p(2) - p(3) + 2*p(1)))/2;
moment_x =  A*r*sqrt(3)*(p(2) - p(3))/2;

%% Moment-only tip wrench

% Wrench convention:
% [Mx; My; Mz; Fx; Fy; Fz]
%
% The axial force is intentionally excluded.
W_pressure = [moment_x;
              moment_y;
              0;
              0;
              0;
              0];

%% Select the configuration used by the Jacobian and gravity model

% Theta is undefined when the arm is straight. Use commanded theta in
% this small region.
if abs(phi_meas) < 1e-6
    theta_for_J = theta_des;
else
    theta_for_J = theta_meas;
end

phi_for_J = phi_meas;

%% Pressure-generated joint torques

J_tip = completeArm_Jacobian( ...
    theta_for_J, phi_for_J, l, N);

tau_pressure_all = J_tip.'*W_pressure;

phi_tau_pressure = zeros(number_phi_joints,1);

for interval = 1:N

    % Columns in the complete 4N-joint Jacobian
    index_all_phi1 = 4*(interval-1) + 2;
    index_all_phi2 = 4*(interval-1) + 3;

    % Locations in the 2N-element output vector
    index_phi1 = 2*interval - 1;
    index_phi2 = 2*interval;

    phi_tau_pressure(index_phi1) = ...
        tau_pressure_all(index_all_phi1);

    phi_tau_pressure(index_phi2) = ...
        tau_pressure_all(index_all_phi2);
end

%% Convert world gravity into the kinematic arm-base frame

% Gravity used in the Simscape Mechanism Configuration block
gravity_world = [0;
                 0;
                -9.80665];

% Fixed alignment between the kinematic frame and the nominal
% horizontal Simscape module frame.
%
% The kinematic arm extends along +z, whereas the horizontal
% Simscape module extends along +y.
R_alignment = [1  0  0;
               0  0  1;
               0 -1  0];       % Rx(-pi/2)

% R_WB is the orientation supplied by the Simscape model.
% Include the fixed initial alignment to obtain the complete
% kinematic-base-to-world rotation.
R_WK = R_WB * R_alignment;

% Express world gravity in the kinematic arm-base frame
gravity_base = R_WK.' * gravity_world;

% Gravity force acting on one disk
gravity_force_disk = disk_mass * gravity_base;

%% Rotation matrices for one rigid-link interval

alpha = phi_for_J/(2*N);

ct = cos(theta_for_J);
st = sin(theta_for_J);

ca = cos(alpha);
sa = sin(alpha);

Rz_theta = [ct, -st, 0;
            st,  ct, 0;
             0,   0, 1];

Rz_minus_theta = [ ct, st, 0;
                   -st, ct, 0;
                     0,  0, 1];

Ry_alpha = [ ca, 0, sa;
              0, 1,  0;
            -sa, 0, ca];

%% Joint axes, joint positions and disk COM positions

joint_axis = zeros(3,number_phi_joints);
joint_position = zeros(3,number_phi_joints);
disk_position = zeros(3,N);

% Pose at the base of the current interval
R_current = eye(3);
position_current = zeros(3,1);

translation_local = [0; 0; l];

for interval = 1:N

    index_phi1 = 2*interval - 1;
    index_phi2 = 2*interval;

    % Apply Rz(theta).
    R_after_theta = R_current*Rz_theta;

    % First phi joint is located at the proximal disk.
    joint_axis(:,index_phi1) = R_after_theta(:,2);
    joint_position(:,index_phi1) = position_current;

    % Apply the first Ry(alpha).
    R_after_phi1 = R_after_theta*Ry_alpha;

    % Translate to the next disk.
    next_disk_position = ...
        position_current + R_after_phi1*translation_local;

    % Second phi joint is located at the distal disk.
    joint_axis(:,index_phi2) = R_after_phi1(:,2);
    joint_position(:,index_phi2) = next_disk_position;

    % Assumption: the disk COM is at the disk-frame origin.
    disk_position(:,interval) = next_disk_position;

    % Complete the interval:
    % Ry(alpha), followed by Rz(-theta).
    R_current = ...
        R_after_phi1*Ry_alpha*Rz_minus_theta;

    position_current = next_disk_position;
end

%% Accumulate downstream gravity forces and moments

% downstream_force(:,i) contains the total gravity force from disk i
% through disk N.
%
% downstream_moment_origin(:,i) contains their total gravity moment
% calculated about the arm-base origin.

downstream_force = zeros(3,N+1);
downstream_moment_origin = zeros(3,N+1);

for disk_number = N:-1:1

    downstream_force(:,disk_number) = ...
        downstream_force(:,disk_number+1) + ...
        gravity_force_disk;

    downstream_moment_origin(:,disk_number) = ...
        downstream_moment_origin(:,disk_number+1) + ...
        cross(disk_position(:,disk_number), ...
              gravity_force_disk);
end

%% Calculate gravity torque at all 58 phi joints

phi_tau_gravity_load = zeros(number_phi_joints,1);

for interval = 1:N

    index_phi1 = 2*interval - 1;
    index_phi2 = 2*interval;

    force_downstream = downstream_force(:,interval);
    moment_downstream_origin = ...
        downstream_moment_origin(:,interval);

    % Gravity moment about the first phi joint
    moment_about_phi1 = ...
        moment_downstream_origin ...
        - cross(joint_position(:,index_phi1), ...
                force_downstream);

    phi_tau_gravity_load(index_phi1) = ...
        joint_axis(:,index_phi1).'*moment_about_phi1;

    % Gravity moment about the second phi joint
    moment_about_phi2 = ...
        moment_downstream_origin ...
        - cross(joint_position(:,index_phi2), ...
                force_downstream);

    phi_tau_gravity_load(index_phi2) = ...
        joint_axis(:,index_phi2).'*moment_about_phi2;
end

%% Gravity compensation

% Gravity compensation acts opposite to the gravity-generated load.
phi_tau_gravity = -phi_tau_gravity_load;

%% Final joint torque commands

% pd_moment_correction is already included in the pressure-generated
% moment. Do not add the same PD output again elsewhere.

% phi_tau = phi_tau_pressure + phi_tau_gravity;

%% Final joint torque commands

% Complete torque vector:
% [Phi1_1; Phi2_1; Phi1_2; Phi2_2; ...]
phi_tau_all = phi_tau_pressure + phi_tau_gravity;

% Temporarily output only the first phi joint in every interval.
phi_tau = phi_tau_all(1:2:end);

end
